simulink model "qs2_pen_ss_model"  (R2023a)
settings: Solver=ode4  StartTime=0.0  StopTime=20  FixedStep=0.002  RelTol=1e-3  EnableMultiTasking=on
values from neighbouring files (symbols this model uses):
  A = zeros(4,4)    [qs2_rotpen_ABCD_eqns_down_student.m]
  B = kt * B / Rm    [qs2_rotpen_ABCD_eqns_down_student.m]
  C = zeros(2,4)    [qs2_rotpen_ABCD_eqns_down_student.m]
  D = zeros(4,1)    [qs2_rotpen_ABCD_eqns_down_student.m]
undefined symbols (not defined in the file or in its folder): HIL, qc_get_step_size
libraries: quarc_library x3
settings Model: SimulationMode=external  ExtModeTrigDuration=10000  Creator=pmartin  LastModifiedBy=dinhck
settings SolverCC: PositivePriorityOrder=on
settings DebuggingCC: UnderspecifiedInitializationDetection=Classic  MergeDetectMultiDrivingBlocksExec=none
settings ModelReferenceCC: PropagateSignalLabelsOutOfModel=off
settings RTWCC: Description=QUARC Win64 Target Using Toolchain  SystemTargetFile=quarc_win64.tlc  Toolchain=QUARC win64 | nmake (64-bit Windows)  BuildConfiguration=Faster Runs
settings STFCustomTargetCC: SystemTargetFile=quarc_win64.tlc
settings GRTTargetCC: ParMdlRefBuildCompliant=off  CompOptLevelCompliant=off  CombineOutputUpdateFcns=off  MatFileLogging=off  CPPClassGenCompliant=off  GRTInterface=on  ExtMode=on  ExtModeMexFile=quarc_comm

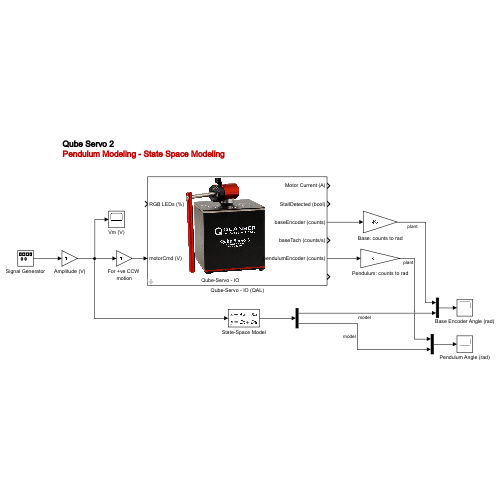
[thumbnail: Simulink's stored preview of the top-level diagram]
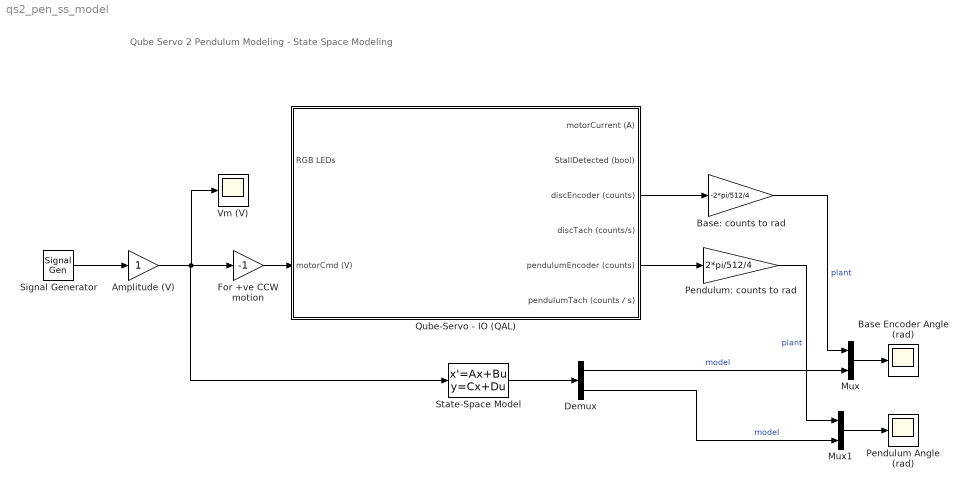
== system qs2_pen_ss_model ==
  note: Qube Servo 2
      | Pendulum Modeling - State Space Modeling
  Amplitude (V) : Gain
  Base Encoder Angle (rad) : Scope
  Base: counts to rad : Gain  Gain=-2*pi/512/4
  Demux : Demux  Outputs=2
  For +ve CCW motion : Gain  Gain=-1
  Mux : Mux  Inputs=2
  Mux1 : Mux  Inputs=2
  Pendulum Angle (rad) : Scope
  Pendulum: counts to rad : Gain  Gain=2*pi/512/4
  Qube-Servo - IO (QAL) : Subsystem  mask{setup=Hardware, top=Pendulum, version=2}
      mask prompts: setup "Qube-Servo Setup:"; top "Qube Add-On:"; version "Qube VERSION"
      mask help:
      | This subsystem provides the core and basic I/O capabilities to read data from and write data to the Qube-Servo 3 using the Quanser HIL API. You can write motor commands and LEDs and read motor current, motor stall detection, and base and pendulum encoder and tachometer.
      |
      | The RGB LEDs command is a 3x1 vector representing,
      | 1. Red LED
      | 2. Green LED
      | 3. Blue LED
      mask init:
      | % if nothing is connected to LED, we read RED which will always be 0 so
      |     % that the qube can turn green okay. Once something is connected, we
      |     % read all rgb channels
      |     blockPortData=get_param(gcb,'PortConnectivity');
      |     if (blockPortData(1).SrcBlock==-1)
      |         set_param([gcb, '/HIL Write'], 'other_channels', '[11000]');
      |     else
      |         set_param([gcb, '/HIL Write'], 'other_channels', '[11000:11002]');
      |     end
      | 
      |     % make sure hil blocks match the hil initialize name
      |     set_param([gcb, '/HIL Write'], 'object_name', get_param([gcb, '/HIL Initialize'], 'object_name'));
      |     set_param([gcb, '/HIL Read Timebase'], 'object_name', get_param([gcb, '/HIL Initialize'], 'object_name'));
      |     
      |     % % make sure board specific options for qube are always set
      |     % set_param([gcb, '/HIL Initialize'], 'board_options', 'deadband_compensation=0.3;pwm_en=0;enc0_velocity=3.0;enc1_velocity=3.0;min_diode_compensation=0.3;max_diode_compensation=1.5');
      |     
      |     % differentiate between hardware and software qubes. Make sure that if
      |     % its hardware, we read both pendulum and disc encoder and tach, even if not
      |     % needed. Hil initialize does not get an ip and port combo. Hil read
      |     % timebase advanced options are set to defaults. 
      |     if strcmp(get_param(gcb, 'version'), '3')
      |         % make sure board specific options for qube are always set
      |         set_param([gcb, '/HIL Initialize'], 'board_options', 'deadband_compensation=0.3;pwm_en=0;enc0_velocity=3.0;enc1_velocity=3.0;min_diode_compensation=0.3;max_diode_compensation=1.5');
      |     
      |         % set_param([gcb, '/HIL Read Timebase'], 'other_channels', '[14000:14001]');
      |         % set for hardware
      |         set_param([gcb, '/HIL Initialize'], 'board_type', 'qube_servo3_usb');
      |         % set_param([gcb, '/HIL Read Timebase'], 'overflow_mode', 'Error on overflow');
      |         % set_param([gcb, '/HIL Read Timebase'], 'samples_in_buffer', 'max(ceil(1/qc_get_step_size), 1)');
      |         % set_param([gcb, '/HIL Write'], 'active', 'OFF');
      |     % if the qube is virtual, the hil read advanced board specific options
      |     % get set to the correct parameters for virtual cars. 
      |     else
      |         % set_param([gcb, '/HIL Read Timebase'], 'overflow_mode', 'Synchronize (for simulated cards only)');
      |         % set_param([gcb, '/HIL Read Timebase'], 'samples_in_buffer', '1');
      |         % set_param([gcb, '/HIL Write'], 'active', 'ON');
      |         set_param([gcb, '/HIL Initialize'], 'board_type', 'qube_servo2_usb');
      |         set_param([gcb, '/HIL Initialize'], 'board_options','');
      |     end
      | 
      |     if strcmp(get_param(gcb, 'setup'), 'Hardware')
      |         if strcmp(get_param(gcb, 'version'), '3')
      |             set_param([gcb, '/HIL Read Timebase'], 'other_channels', '[14000:14001]');
      |         else
      |             set_param([gcb, '/HIL Read Timebase'], 'other_channels', '[14000]');
      |         end
      |         % set for hardware
      |         set_param([gcb, '/HIL Initialize'], 'board_number', '0');
      |         set_param([gcb, '/HIL Read Timebase'], 'overflow_mode', 'Error on overflow');
      |         set_param([gcb, '/HIL Read Timebase'], 'samples_in_buffer', 'max(ceil(1/qc_get_step_size), 1)');
      |         set_param([gcb, '/HIL Write'], 'active', 'OFF');
      |     % if the qube is virtual, the hil read advanced board specific options
      |     % get set to the correct parameters for virtual cars. 
      |     else
      |         set_param([gcb, '/HIL Read Timebase'], 'overflow_mode', 'Synchronize (for simulated cards only)');
      |         set_param([gcb, '/HIL Read Timebase'], 'samples_in_buffer', '1');
      |         set_param([gcb, '/HIL Write'], 'active', 'ON');
      |     end
      | 
      |     % if set up tach ports for virtual disc vs pendulum. Virtual disc does not support the existence of
      |     % pendulum tach. Also sets up ip and portnumber in the hil initialize. 
      |     if strcmp(get_param(gcb, 'setup'), 'Virtual') && strcmp(get_param(gcb, 'top'), 'Disc')
      |         set_param([gcb, '/HIL Initialize'], 'board_number', '0@tcpip://localhost:18922');
      |         
      |     elseif strcmp(get_param(gcb, 'setup'), 'Virtual') && strcmp(get_param(gcb, 'top'), 'Pendulum')
      |         set_param([gcb, '/HIL Initialize'], 'board_number', '0@tcpip://localhost:18923');
      |         set_param([gcb, '/HIL Read Timebase'], 'other_channels', '[14000:14001]');
      |     end 
      | 
      |     pendulum_encoder_name = 'pendulumEncoder (counts)';
      |     pendulum_encoder = [gcb,'/',pendulum_encoder_name];
      |     
      |     pendulum_tach_name = 'pendulumTach (counts／s)';
      |     pendulum_tach = [gcb,'/',pendulum_tach_name];
      |     
      |     timebase_name = 'HIL Read Timebase';
      |     
      |     % create pendulum encoder and pendulum tach ports and connections if
      |     % needed. Delete them if using the disc. 
      |     if strcmp(get_param(gcb, 'top'), 'Pendulum')
      |         if isempty(find_system(gcbh,'LookUnderMasks','all','Name',pendulum_encoder_name))
      |             add_block('built-in/Outport',pendulum_encoder, 'Port','5','Position',[1050,568,1080,582]);
      |             add_line(gcbh,[timebase_name,'/3'],[pendulum_encoder_name,'/1'],'autorouting','on');
      |         end
      |         if isempty(find_system(gcbh,'LookUnderMasks','all','Name',pendulum_tach_name))
      |             add_block('built-in/Outport',pendulum_tach, 'Port','6','Position',[1050, 603, 1080,617]);
      |             add_line(gcbh,[timebase_name,'/6'],[pendulum_tach_name,'/1'],'autorouting','on');
      |         end 
      |     
      |     else
      |         if ~isempty(find_system(gcbh,'LookUnderMasks','all','Name',pendulum_encoder_name))
      |             delete_line(gcbh,[timebase_name,'/3'],[pendulum_encoder_name,'/1']);
      |             delete_block(pendulum_encoder);
      |         end
      |         if ~isempty(find_system(gcbh,'LookUnderMasks','all','Name',pendulum_tach_name))
      |             delete_line(gcbh,[timebase_name,'/6'],[pendulum_tach_name,'/1']);
      |             delete_block(pendulum_tach);
      |         end 
      |     end
      | 
      |     if strcmp(get_param(gcb, 'setup'), 'Virtual') && strcmp(get_param(gcb, 'top'), 'Disc')
      |         set_param([gcb, '/HIL Read Timebase'], 'other_channels', '[14000]');
      |     end
      settings: CopyFcn=set_param(gcbh,'LinkStatus','none');
      mask TypeOptions setup: Hardware | Virtual
      mask TypeOptions top: Disc | Pendulum
      mask TypeOptions version: 2 | 3
      mask Display:
      | ud = get_param(gcb,'UserData');
      | if (strcmp(get_param(gcb, 'top'), 'Disc') && strcmp(get_param(gcb, 'setup'), 'Hardware'))
      |     image(ud.hardwareDisc);
      | elseif (strcmp(get_param(gcb, 'top'), 'Pendulum') && strcmp(get_param(gcb, 'setup'), 'Hardware'))
      |     image(ud.hardwarePendulum);
      | elseif (strcmp(get_param(gcb, 'top'), 'Disc') && strcmp(get_param(gcb, 'setup'), 'Virtual'))
      |     image(ud.virtualDisc);
      | else
      |     image(ud.virtualPendulum);
      | end
      | 
      | text(.3,.05,'Qube-Servo - IO');
      | 
      | if strcmp(get_param(gcb, 'top'), 'Pendulum')
      |     port_label('input', 1, 'RGB LEDs (%)');
      |     port_label('input', 2, 'motorCmd (V)');
      |     port_label('output', 1, 'Motor Current (A)');
      |     port_label('output', 2, 'StallDetected (bool)');
      |     port_label('output', 3, 'baseEncoder (counts)');
      |     port_label('output', 4, 'baseTach (counts/s)');
      |     port_label('output', 5, 'pendulumEncoder (counts)');
      |     if strcmp(get_param(gcb, 'version'), '3')
      |         port_label('output', 6, 'pendulumTach (counts/s)');
      |     % else
      |     %     set_param([gcb, '/HIL Read Timebase'], 'other_channels', '[14000]');
      |     end
      |     % port_label('output', 6, 'pendulumTach (counts/s)');
      | 
      | else
      |     port_label('input', 1, 'RGB LEDs (%)');
      |     port_label('input', 2, 'motorCmd (V)');
      |     port_label('output', 1, 'Motor Current (A)');
      |     port_label('output', 2, 'StallDetected (bool)');
      |     port_label('output', 3, 'baseEncoder (counts)');
      |     port_label('output', 4, 'baseTach (counts/s)');
      | end
  Signal Generator : SignalGenerator  WaveForm=square
  State-Space Model : StateSpace  A=A  B=B  C=C  D=D  InitialCondition=[0 0 0 0]
  Vm (V) : Scope
  wires:
  State-Space Model/1 -> Demux/1
  Mux/1 -> Base Encoder Angle (rad)/1
  Mux1/1 -> Pendulum Angle (rad)/1
  Base: counts to rad/1 -> Mux/1  "plant"
  Pendulum: counts to rad/1 -> Mux1/1  "plant"
  Demux/1 -> Mux/2  "model"
  Demux/2 -> Mux1/2  "model"
  Amplitude (V)/1 -> State-Space Model/1, Vm (V)/1, For +ve CCW motion/1
  Signal Generator/1 -> Amplitude (V)/1
  Qube-Servo - IO (QAL)/3(discEncoder (counts)) -> Base: counts to rad/1
  Qube-Servo - IO (QAL)/5(pendulumEncoder (counts)) -> Pendulum: counts to rad/1
  For +ve CCW motion/1 -> Qube-Servo - IO (QAL)/2(motorCmd (V))

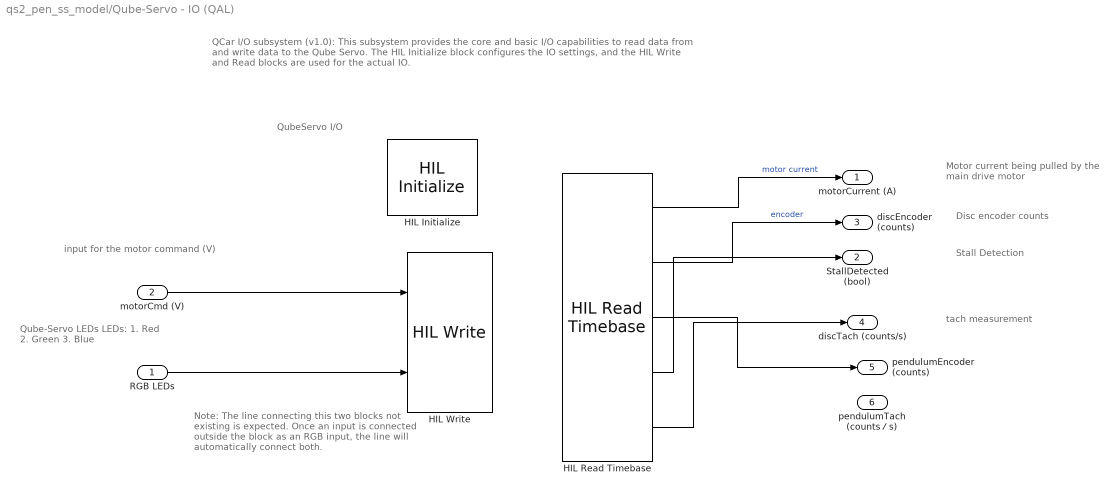
== system qs2_pen_ss_model/Qube-Servo - IO (QAL) ==
  note: Motor current being pulled by the main drive motor
  note: Stall Detection
  note: tach measurement
  note: Disc encoder counts
  note: input for the motor command (V)
  note: QCar I/O subsystem (v1.0):
      |
      | This subsystem provides the core and basic I/O capabilities to read data from and write data to the Qube Servo. The HIL Initialize block configures the IO settings, and the HIL Write and Read blocks are used for the actual IO.
  note: QubeServo I/O
  note: Qube-Servo LEDs
      |
      | LEDs:
      | 1. Red
      | 2. Green
      | 3. Blue
  note: Note: The line connecting this two blocks
      | not existing is expected.
      | Once an input is connected outside the block
      | as an RGB input, the line will automatically
      | connect both.
  RGB LEDs : Inport
  motorCmd (V) : Inport  Port=2
  HIL Initialize : quarc_library/Data Acquisition/Generic/Configuration/HIL Initialize  object_name=HIL-2  board_type=qube_servo2_usb  board_number=0  exclusive=off  active=on  hardware_clocks=[0]  clock_modes=[]  initial_clock_frequencies=[]  set_clock_params_at_start=off  set_clock_params_at_switch_in=off  set_clock_frequencies_at_start=off  set_clock_frequencies_at_switch_in=off  analog_input_channels=[0]  analog_input_configurations=[]  analog_input_maximums=3  analog_input_minimums=-3  set_analog_input_params_at_start=off  set_analog_input_params_at_switch_in=off  analog_output_channels=[0]  analog_output_maximums=15  analog_output_minimums=-15  initial_analog_outputs=[0]  final_analog_outputs=[0]  watchdog_analog_outputs=0  set_analog_output_params_at_start=off  set_analog_output_params_at_switch_in=off  set_analog_outputs_at_start=on  set_analog_outputs_at_switch_in=off  set_analog_outputs_at_terminate=on  set_analog_outputs_at_switch_out=off  set_analog_outputs_on_watchdog=on  digital_input_channels=[]  digital_output_channels=[0]  digital_output_configuration=[]  initial_digital_outputs=[1]  final_digital_outputs=[0]  watchdog_digital_outputs=[0]  set_digital_output_params_at_start=off  set_digital_output_params_at_switch_in=off  set_digital_outputs_at_start=on  set_digital_outputs_at_switch_in=off  set_digital_outputs_at_terminate=on  set_digital_outputs_at_switch_out=off  set_digital_outputs_on_watchdog=on  encoder_channels=[0:1]  quadrature=[4]  encoder_filter_frequency=[]  initial_encoder_counts=[0]  set_encoder_params_at_start=off  set_encoder_params_at_switch_in=off  set_encoder_counts_at_start=on  set_encoder_counts_at_switch_in=off  pwm_channels=[]  pwm_modes=[0]  pwm_frequency=23195  pwm_configuration=[1]  pwm_alignment=[0]  pwm_polarity=[1]  pwm_leading_deadband=[0]  pwm_trailing_deadband=[0]  initial_pwm_outputs=[0]  final_pwm_outputs=[0]  watchdog_pwm_outputs=[]  set_pwm_params_at_start=off  set_pwm_params_at_switch_in=off  set_pwm_outputs_at_start=off  set_pwm_outputs_at_switch_in=off  set_pwm_outputs_at_terminate=off  set_pwm_outputs_at_switch_out=off  set_pwm_outputs_on_watchdog=off  other_output_channels=[11000:11002]  initial_other_outputs=[0 1 0]  final_other_outputs=[1 0 0]  watchdog_other_outputs=[0 0 1]  set_other_outputs_at_start=on  set_other_outputs_at_switch_in=off  set_other_outputs_at_terminate=on  set_other_outputs_at_switch_out=off  set_other_outputs_on_watchdog=on
  HIL Read Timebase : quarc_library/Data Acquisition/Generic/Timebases/HIL Read Timebase  object_name=HIL-2  clock=0  analog_channels=[0]  encoder_channels=[0:1]  digital_channels=[1]  other_channels=[14000]  active=on  vector_output=off  data_type_mode=Inherit via back propagation  encoder_data_type=double  digital_data_type=boolean  overflow_mode=Error on overflow  samples_in_buffer=max(ceil(1/qc_get_step_size), 1)
  HIL Write : quarc_library/Data Acquisition/Generic/Immediate I//O/HIL Write  object_name=HIL-2  analog_channels=[0]  pwm_channels=[]  digital_channels=[]  other_channels=[11000]  sample_time=-1  active=off  vector_input=on
  motorCurrent (A) : Outport  VectorParamsAs1DForOutWhenUnconnected=off
  StallDetected (bool) : Outport  Port=2  VectorParamsAs1DForOutWhenUnconnected=off
  discEncoder (counts) : Outport  Port=3  VectorParamsAs1DForOutWhenUnconnected=off
  discTach (counts/s) : Outport  Port=4  VectorParamsAs1DForOutWhenUnconnected=off
  pendulumEncoder (counts) : Outport  Port=5
  pendulumTach (counts／s) : Outport  Port=6
  wires:
  RGB LEDs/1 -> HIL Write/2
  HIL Read Timebase/5 -> discTach (counts/s)/1
  HIL Read Timebase/2 -> discEncoder (counts)/1  "encoder"
  HIL Read Timebase/4 -> StallDetected (bool)/1
  HIL Read Timebase/1 -> motorCurrent (A)/1  "motor current"
  motorCmd (V)/1 -> HIL Write/1
  HIL Read Timebase/3 -> pendulumEncoder (counts)/1
  ? -> pendulumTach (counts／s)/1
